simulink model "BehProductionCell"  (R2026b)
settings: Solver=VariableStepAuto
model workspace (MAT data in the model file):
  CellBatchSize_bowls = 40
  CellCalibPeriod_s = 5400
  CellCalibTime_s = 90
  CellCleanTime_s = 120
  CellDrainTime_s = 150
  CellFillRate_bps = 0.4
  CellHeaterPower_kW = 32
  CellPackRate_bph = 85
  CellPrepRate_bph = 80
  CellQCRate_bph = 90
  CellRejectFrac = 0.02
  CellSimmerTime_s = 1182
  CellVatThermalMass_JpK = 96000
settings Model: DataDictionary=BehParamsCommon.sldd  ParameterArgumentNames=CellPrepRate_bph,CellBatchSize_bowls,CellHeaterPower_kW,CellVatThermalMass_JpK,CellFillRate_bps,CellSimmerTime_s,CellDrainTime_s,CellCleanTime_s,CellQCRate_bph,CellRejectFrac,CellCalibPeriod_s,CellCalibTime_s,CellPackRate_bph  Creator=sarah  LastModifiedBy=sdagen

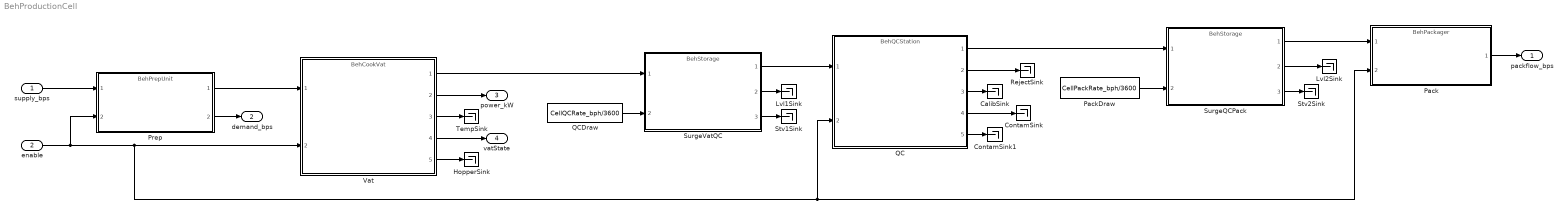
== system BehProductionCell ==
  supply_bps : Inport
  enable : Inport  Port=2
  CalibSink : Terminator
  ContamSink : Terminator
  ContamSink1 : Terminator
  HopperSink : Terminator
  Lvl1Sink : Terminator
  Lvl2Sink : Terminator
  Pack : ModelReference  ModelNameDialog=BehPackager  UsingDefaultArgumentValue=0,0  SimulationMode=Normal  ModelReferenceVersion=1.5
  PackDraw : Constant  Value=CellPackRate_bph/3600
  Prep : ModelReference  ModelNameDialog=BehPrepUnit  UsingDefaultArgumentValue=0,0  SimulationMode=Normal  ModelReferenceVersion=1.5
  QC : ModelReference  ModelNameDialog=BehQCStation  UsingDefaultArgumentValue=0,0,0,0,0,0  SimulationMode=Normal  ModelReferenceVersion=1.6
  QCDraw : Constant  Value=CellQCRate_bph/3600
  RejectSink : Terminator
  Stv1Sink : Terminator
  Stv2Sink : Terminator
  SurgeQCPack : ModelReference  ModelNameDialog=BehStorage  UsingDefaultArgumentValue=0,0  SimulationMode=Normal  ModelReferenceVersion=1.5
  SurgeVatQC : ModelReference  ModelNameDialog=BehStorage  UsingDefaultArgumentValue=0,0  SimulationMode=Normal  ModelReferenceVersion=1.5
  TempSink : Terminator
  Vat : ModelReference  ModelNameDialog=BehCookVat  UsingDefaultArgumentValue=0,0,0,0,0,0,0,0  SimulationMode=Normal  ModelReferenceVersion=1.16
  packflow_bps : Outport
  demand_bps : Outport  Port=2
  power_kW : Outport  Port=3
  vatState : Outport  Port=4
  wires:
  QC/1 -> SurgeQCPack/1
  QCDraw/1 -> SurgeVatQC/2
  supply_bps/1 -> Prep/1
  Prep/2 -> demand_bps/1
  PackDraw/1 -> SurgeQCPack/2
  Prep/1 -> Vat/1
  enable/1 -> Pack/2, QC/2, Vat/2, Prep/2
  SurgeVatQC/3 -> Stv1Sink/1
  Vat/3 -> TempSink/1
  SurgeVatQC/2 -> Lvl1Sink/1
  Vat/2 -> power_kW/1
  SurgeQCPack/3 -> Stv2Sink/1
  SurgeVatQC/1 -> QC/1
  Vat/1 -> SurgeVatQC/1
  Vat/4 -> vatState/1
  Vat/5 -> HopperSink/1
  QC/2 -> RejectSink/1
  SurgeQCPack/1 -> Pack/1
  QC/3 -> CalibSink/1
  SurgeQCPack/2 -> Lvl2Sink/1
  Pack/1 -> packflow_bps/1
  QC/4 -> ContamSink/1
  QC/5 -> ContamSink1/1
